simulink library "Batteries"  (R2025b)
settings: Solver=VariableStepAuto  StartTime=0.0  StopTime=10.0  RelTol=1e-3
undefined symbols (not defined in the file or in its folder): battery_builder_rtmsupport, gcbh
libraries: Batteries_lib x12
(part 2 of 2)

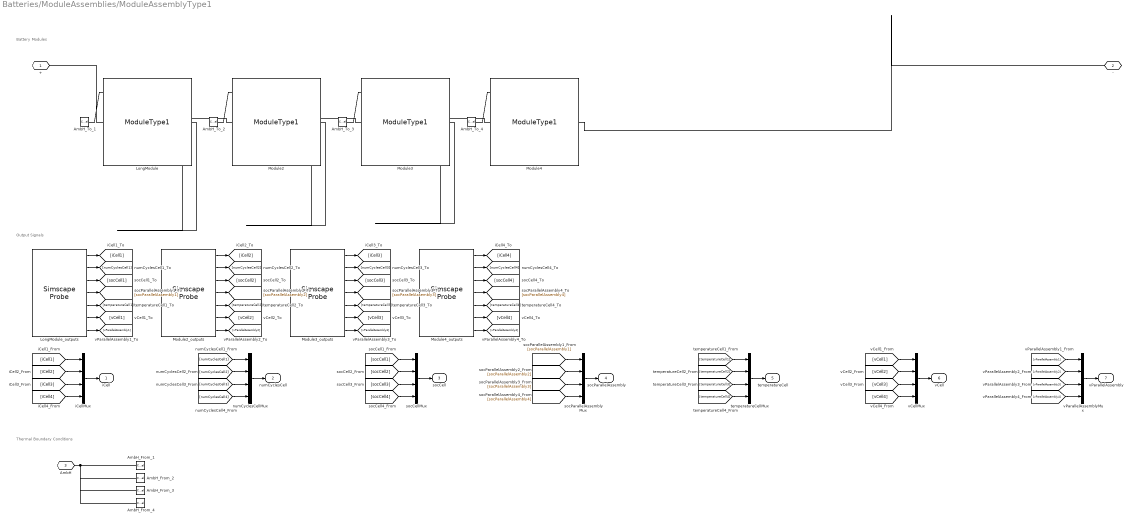
== system Batteries/ModuleAssemblies/ModuleAssemblyType1 ==
  note: Battery Modules
  note: Output Signals
  note: Thermal Boundary Conditions
  AmbH_From_1 : ConnectionLabel  Label=ambH_1
  AmbH_From_2 : ConnectionLabel  Label=ambH_2
  AmbH_From_3 : ConnectionLabel  Label=ambH_3
  AmbH_From_4 : ConnectionLabel  Label=ambH_4
  AmbH_To_1 : ConnectionLabel  Label=ambH_1
  AmbH_To_2 : ConnectionLabel  Label=ambH_2
  AmbH_To_3 : ConnectionLabel  Label=ambH_3
  AmbH_To_4 : ConnectionLabel  Label=ambH_4
  LongModule : Batteries_lib/Modules/ModuleType1  SOC_vecCell=[0, .1, .25, .5, .75, .9, 1]  T_vecCell=[278, 293, 313] K  V0_matCell=[3.49, 3.5, 3.51; 3.55, 3.57, 3.56; 3.62, 3.63, 3.64; 3.71, 3.71, 3.72; 3.91, 3.93, 3.94; 4.07, 4.08, 4.08; 4.19, 4.19, 4.19] V  V_rangeCell=[0, inf] V  R0_matCell=[.0117, .0085, .009; .011, .0085, .009; .0114, .0087, .0092; .0107, .0082, .0088; .0107, .0083, .0091; .0113, .0085, .0089; .0116, .0085, .0089] Ohm  AHCell=27 A*hr  extrapolation_optionCell=simscape.enum.extrapolation.nearest  thermal_massCell=100 J/K  CoolantResistance=1.2 K/W  AmbientResistance=25 K/W  P=20  S=2  iCell_specify=off  iCell_priority=None  iCell=0 A  iCell_nominal_specify=off  iCell_nominal_value=1  iCell_nominal_unit=A  vCell_specify=off  vCell_priority=None  vCell=0 V  vCell_nominal_specify=off  vCell_nominal_value=1  vCell_nominal_unit=V  socCell_specify=off  socCell_priority=High  socCell=1  socCell_nominal_specify=off  socCell_nominal_value=1  socCell_nominal_unit=1  numCyclesCell_specify=off  numCyclesCell_priority=High  numCyclesCell=0  numCyclesCell_nominal_specify=off  numCyclesCell_nominal_value=1  numCyclesCell_nominal_unit=1  temperatureCell_specify=off  temperatureCell_priority=High  temperatureCell=298.15 K  temperatureCell_nominal_specify=off  temperatureCell_nominal_value=1  temperatureCell_nominal_unit=K  vParallelAssembly_specify=off  vParallelAssembly_priority=None  vParallelAssembly=repmat(0, 2, 1) V  vParallelAssembly_nominal_specify=off  vParallelAssembly_nominal_value=1  vParallelAssembly_nominal_unit=V  socParallelAssembly_specify=off  socParallelAssembly_priority=None  socParallelAssembly=repmat(1, 2, 1)  socParallelAssembly_nominal_specify=off  socParallelAssembly_nominal_value=1  socParallelAssembly_nominal_unit=1
      settings: InternalSimscapePortConfiguration="{\"Bottom\":[{\"id\":\"n\",\"label\":\"-\",\"type\":\"foundation.electrical.electrical\"}],\"Left\":[{\"id\":\"AmbH\",\"label\":\"AmbH\",\"type\":\"foundation.thermal.thermal\"}],\"Right\":[],\"Top\":[{\"id\":\"p\",\"label\":\"+\",\"type\":\"foundation.electrical.electrical\"},{\"id\":\"TopExtClnt\",\"label\":\"CPT\",\"type\":\"foundation.thermal.thermal\"}]}"
  LongModule_outputs : SimscapeProbe  BoundBlock=3  Variables="{\"iCell\":{\"Probing\":\"ON\"},\"numCyclesCell\":{\"Probing\":\"ON\"},\"socCell\":{\"Probing\":\"ON\"},\"socParallelAssembly\":{\"Probing\":\"ON\"},\"temperatureCell\":{\"Probing\":\"ON\"},\"vCell\":{\"Probing\":\"ON\"},\"vParallelAssembly\":{\"Probing\":\"ON\"}}"
  Module2 : Batteries_lib/Modules/ModuleType1  SOC_vecCell=[0, .1, .25, .5, .75, .9, 1]  T_vecCell=[278, 293, 313] K  V0_matCell=[3.49, 3.5, 3.51; 3.55, 3.57, 3.56; 3.62, 3.63, 3.64; 3.71, 3.71, 3.72; 3.91, 3.93, 3.94; 4.07, 4.08, 4.08; 4.19, 4.19, 4.19] V  V_rangeCell=[0, inf] V  R0_matCell=[.0117, .0085, .009; .011, .0085, .009; .0114, .0087, .0092; .0107, .0082, .0088; .0107, .0083, .0091; .0113, .0085, .0089; .0116, .0085, .0089] Ohm  AHCell=27 A*hr  extrapolation_optionCell=simscape.enum.extrapolation.nearest  thermal_massCell=100 J/K  CoolantResistance=1.2 K/W  AmbientResistance=25 K/W  P=20  S=2  iCell_specify=off  iCell_priority=None  iCell=0 A  iCell_nominal_specify=off  iCell_nominal_value=1  iCell_nominal_unit=A  vCell_specify=off  vCell_priority=None  vCell=0 V  vCell_nominal_specify=off  vCell_nominal_value=1  vCell_nominal_unit=V  socCell_specify=off  socCell_priority=High  socCell=1  socCell_nominal_specify=off  socCell_nominal_value=1  socCell_nominal_unit=1  numCyclesCell_specify=off  numCyclesCell_priority=High  numCyclesCell=0  numCyclesCell_nominal_specify=off  numCyclesCell_nominal_value=1  numCyclesCell_nominal_unit=1  temperatureCell_specify=off  temperatureCell_priority=High  temperatureCell=298.15 K  temperatureCell_nominal_specify=off  temperatureCell_nominal_value=1  temperatureCell_nominal_unit=K  vParallelAssembly_specify=off  vParallelAssembly_priority=None  vParallelAssembly=repmat(0, 2, 1) V  vParallelAssembly_nominal_specify=off  vParallelAssembly_nominal_value=1  vParallelAssembly_nominal_unit=V  socParallelAssembly_specify=off  socParallelAssembly_priority=None  socParallelAssembly=repmat(1, 2, 1)  socParallelAssembly_nominal_specify=off  socParallelAssembly_nominal_value=1  socParallelAssembly_nominal_unit=1
      settings: InternalSimscapePortConfiguration="{\"Bottom\":[{\"id\":\"n\",\"label\":\"-\",\"type\":\"foundation.electrical.electrical\"}],\"Left\":[{\"id\":\"AmbH\",\"label\":\"AmbH\",\"type\":\"foundation.thermal.thermal\"}],\"Right\":[],\"Top\":[{\"id\":\"p\",\"label\":\"+\",\"type\":\"foundation.electrical.electrical\"},{\"id\":\"TopExtClnt\",\"label\":\"CPT\",\"type\":\"foundation.thermal.thermal\"}]}"
  Module2_outputs : SimscapeProbe  BoundBlock=4  Variables="{\"iCell\":{\"Probing\":\"ON\"},\"numCyclesCell\":{\"Probing\":\"ON\"},\"socCell\":{\"Probing\":\"ON\"},\"socParallelAssembly\":{\"Probing\":\"ON\"},\"temperatureCell\":{\"Probing\":\"ON\"},\"vCell\":{\"Probing\":\"ON\"},\"vParallelAssembly\":{\"Probing\":\"ON\"}}"
  Module3 : Batteries_lib/Modules/ModuleType1  SOC_vecCell=[0, .1, .25, .5, .75, .9, 1]  T_vecCell=[278, 293, 313] K  V0_matCell=[3.49, 3.5, 3.51; 3.55, 3.57, 3.56; 3.62, 3.63, 3.64; 3.71, 3.71, 3.72; 3.91, 3.93, 3.94; 4.07, 4.08, 4.08; 4.19, 4.19, 4.19] V  V_rangeCell=[0, inf] V  R0_matCell=[.0117, .0085, .009; .011, .0085, .009; .0114, .0087, .0092; .0107, .0082, .0088; .0107, .0083, .0091; .0113, .0085, .0089; .0116, .0085, .0089] Ohm  AHCell=27 A*hr  extrapolation_optionCell=simscape.enum.extrapolation.nearest  thermal_massCell=100 J/K  CoolantResistance=1.2 K/W  AmbientResistance=25 K/W  P=20  S=2  iCell_specify=off  iCell_priority=None  iCell=0 A  iCell_nominal_specify=off  iCell_nominal_value=1  iCell_nominal_unit=A  vCell_specify=off  vCell_priority=None  vCell=0 V  vCell_nominal_specify=off  vCell_nominal_value=1  vCell_nominal_unit=V  socCell_specify=off  socCell_priority=High  socCell=1  socCell_nominal_specify=off  socCell_nominal_value=1  socCell_nominal_unit=1  numCyclesCell_specify=off  numCyclesCell_priority=High  numCyclesCell=0  numCyclesCell_nominal_specify=off  numCyclesCell_nominal_value=1  numCyclesCell_nominal_unit=1  temperatureCell_specify=off  temperatureCell_priority=High  temperatureCell=298.15 K  temperatureCell_nominal_specify=off  temperatureCell_nominal_value=1  temperatureCell_nominal_unit=K  vParallelAssembly_specify=off  vParallelAssembly_priority=None  vParallelAssembly=repmat(0, 2, 1) V  vParallelAssembly_nominal_specify=off  vParallelAssembly_nominal_value=1  vParallelAssembly_nominal_unit=V  socParallelAssembly_specify=off  socParallelAssembly_priority=None  socParallelAssembly=repmat(1, 2, 1)  socParallelAssembly_nominal_specify=off  socParallelAssembly_nominal_value=1  socParallelAssembly_nominal_unit=1
      settings: InternalSimscapePortConfiguration="{\"Bottom\":[{\"id\":\"n\",\"label\":\"-\",\"type\":\"foundation.electrical.electrical\"}],\"Left\":[{\"id\":\"AmbH\",\"label\":\"AmbH\",\"type\":\"foundation.thermal.thermal\"}],\"Right\":[],\"Top\":[{\"id\":\"p\",\"label\":\"+\",\"type\":\"foundation.electrical.electrical\"},{\"id\":\"TopExtClnt\",\"label\":\"CPT\",\"type\":\"foundation.thermal.thermal\"}]}"
  Module3_outputs : SimscapeProbe  BoundBlock=5  Variables="{\"iCell\":{\"Probing\":\"ON\"},\"numCyclesCell\":{\"Probing\":\"ON\"},\"socCell\":{\"Probing\":\"ON\"},\"socParallelAssembly\":{\"Probing\":\"ON\"},\"temperatureCell\":{\"Probing\":\"ON\"},\"vCell\":{\"Probing\":\"ON\"},\"vParallelAssembly\":{\"Probing\":\"ON\"}}"
  Module4 : Batteries_lib/Modules/ModuleType1  SOC_vecCell=[0, .1, .25, .5, .75, .9, 1]  T_vecCell=[278, 293, 313] K  V0_matCell=[3.49, 3.5, 3.51; 3.55, 3.57, 3.56; 3.62, 3.63, 3.64; 3.71, 3.71, 3.72; 3.91, 3.93, 3.94; 4.07, 4.08, 4.08; 4.19, 4.19, 4.19] V  V_rangeCell=[0, inf] V  R0_matCell=[.0117, .0085, .009; .011, .0085, .009; .0114, .0087, .0092; .0107, .0082, .0088; .0107, .0083, .0091; .0113, .0085, .0089; .0116, .0085, .0089] Ohm  AHCell=27 A*hr  extrapolation_optionCell=simscape.enum.extrapolation.nearest  thermal_massCell=100 J/K  CoolantResistance=1.2 K/W  AmbientResistance=25 K/W  P=20  S=2  iCell_specify=off  iCell_priority=None  iCell=0 A  iCell_nominal_specify=off  iCell_nominal_value=1  iCell_nominal_unit=A  vCell_specify=off  vCell_priority=None  vCell=0 V  vCell_nominal_specify=off  vCell_nominal_value=1  vCell_nominal_unit=V  socCell_specify=off  socCell_priority=High  socCell=1  socCell_nominal_specify=off  socCell_nominal_value=1  socCell_nominal_unit=1  numCyclesCell_specify=off  numCyclesCell_priority=High  numCyclesCell=0  numCyclesCell_nominal_specify=off  numCyclesCell_nominal_value=1  numCyclesCell_nominal_unit=1  temperatureCell_specify=off  temperatureCell_priority=High  temperatureCell=298.15 K  temperatureCell_nominal_specify=off  temperatureCell_nominal_value=1  temperatureCell_nominal_unit=K  vParallelAssembly_specify=off  vParallelAssembly_priority=None  vParallelAssembly=repmat(0, 2, 1) V  vParallelAssembly_nominal_specify=off  vParallelAssembly_nominal_value=1  vParallelAssembly_nominal_unit=V  socParallelAssembly_specify=off  socParallelAssembly_priority=None  socParallelAssembly=repmat(1, 2, 1)  socParallelAssembly_nominal_specify=off  socParallelAssembly_nominal_value=1  socParallelAssembly_nominal_unit=1
      settings: InternalSimscapePortConfiguration="{\"Bottom\":[{\"id\":\"n\",\"label\":\"-\",\"type\":\"foundation.electrical.electrical\"}],\"Left\":[{\"id\":\"AmbH\",\"label\":\"AmbH\",\"type\":\"foundation.thermal.thermal\"}],\"Right\":[],\"Top\":[{\"id\":\"p\",\"label\":\"+\",\"type\":\"foundation.electrical.electrical\"},{\"id\":\"TopExtClnt\",\"label\":\"CPT\",\"type\":\"foundation.thermal.thermal\"}]}"
  Module4_outputs : SimscapeProbe  BoundBlock=6  Variables="{\"iCell\":{\"Probing\":\"ON\"},\"numCyclesCell\":{\"Probing\":\"ON\"},\"socCell\":{\"Probing\":\"ON\"},\"socParallelAssembly\":{\"Probing\":\"ON\"},\"temperatureCell\":{\"Probing\":\"ON\"},\"vCell\":{\"Probing\":\"ON\"},\"vParallelAssembly\":{\"Probing\":\"ON\"}}"
  iCellMux : Mux
  numCyclesCellMux : Mux
  socCellMux : Mux
  socParallelAssemblyMux : Mux
  temperatureCellMux : Mux
  vCellMux : Mux
  vParallelAssemblyMux : Mux
  + : PMIOPort  Side=Left
  - : PMIOPort  Port=2  Side=Right
  AmbH : PMIOPort  Port=3  Side=Right  ConnectionType=Connection: foundation.thermal.thermal
  iCell : Outport
  numCyclesCell : Outport  Port=2
  socCell : Outport  Port=3
  socParallelAssembly : Outport  Port=4
  temperatureCell : Outport  Port=5
  vCell : Outport  Port=6
  vParallelAssembly : Outport  Port=7
  wires:
  LongModule_outputs/1 -> [iCell1]
  iCellMux/1 -> iCell/1
  [iCell1] -> iCellMux/1
  LongModule_outputs/2 -> [numCyclesCell1]
  numCyclesCellMux/1 -> numCyclesCell/1
  [numCyclesCell1] -> numCyclesCellMux/1
  LongModule_outputs/3 -> [socCell1]
  socCellMux/1 -> socCell/1
  [socCell1] -> socCellMux/1
  LongModule_outputs/4 -> [socParallelAssembly1]
  socParallelAssemblyMux/1 -> socParallelAssembly/1
  [socParallelAssembly1] -> socParallelAssemblyMux/1
  LongModule_outputs/5 -> [temperatureCell1]
  temperatureCellMux/1 -> temperatureCell/1
  [temperatureCell1] -> temperatureCellMux/1
  LongModule_outputs/6 -> [vCell1]
  vCellMux/1 -> vCell/1
  [vCell1] -> vCellMux/1
  LongModule_outputs/7 -> [vParallelAssembly1]
  vParallelAssemblyMux/1 -> vParallelAssembly/1
  [vParallelAssembly1] -> vParallelAssemblyMux/1
  Module2_outputs/1 -> [iCell2]
  [iCell2] -> iCellMux/2
  Module2_outputs/2 -> [numCyclesCell2]
  [numCyclesCell2] -> numCyclesCellMux/2
  Module2_outputs/3 -> [socCell2]
  [socCell2] -> socCellMux/2
  Module2_outputs/4 -> [socParallelAssembly2]
  [socParallelAssembly2] -> socParallelAssemblyMux/2
  Module2_outputs/5 -> [temperatureCell2]
  [temperatureCell2] -> temperatureCellMux/2
  Module2_outputs/6 -> [vCell2]
  [vCell2] -> vCellMux/2
  Module2_outputs/7 -> [vParallelAssembly2]
  [vParallelAssembly2] -> vParallelAssemblyMux/2
  Module3_outputs/1 -> [iCell3]
  [iCell3] -> iCellMux/3
  Module3_outputs/2 -> [numCyclesCell3]
  [numCyclesCell3] -> numCyclesCellMux/3
  Module3_outputs/3 -> [socCell3]
  [socCell3] -> socCellMux/3
  Module3_outputs/4 -> [socParallelAssembly3]
  [socParallelAssembly3] -> socParallelAssemblyMux/3
  Module3_outputs/5 -> [temperatureCell3]
  [temperatureCell3] -> temperatureCellMux/3
  Module3_outputs/6 -> [vCell3]
  [vCell3] -> vCellMux/3
  Module3_outputs/7 -> [vParallelAssembly3]
  [vParallelAssembly3] -> vParallelAssemblyMux/3
  Module4_outputs/1 -> [iCell4]
  [iCell4] -> iCellMux/4
  Module4_outputs/2 -> [numCyclesCell4]
  [numCyclesCell4] -> numCyclesCellMux/4
  Module4_outputs/3 -> [socCell4]
  [socCell4] -> socCellMux/4
  Module4_outputs/4 -> [socParallelAssembly4]
  [socParallelAssembly4] -> socParallelAssemblyMux/4
  Module4_outputs/5 -> [temperatureCell4]
  [temperatureCell4] -> temperatureCellMux/4
  Module4_outputs/6 -> [vCell4]
  [vCell4] -> vCellMux/4
  Module4_outputs/7 -> [vParallelAssembly4]
  [vParallelAssembly4] -> vParallelAssemblyMux/4
  connections:
  Module2/LConn2 -- LongModule/RConn1
  Module3/LConn2 -- Module2/RConn1
  Module4/LConn2 -- Module3/RConn1
  LongModule/LConn2 -- +/RConn1
  Module4/RConn1 -- -/RConn1
  AmbH_To_1/LConn1 -- LongModule/LConn1
  AmbH_From_1/LConn1 -- AmbH_From_2/LConn1 -- AmbH_From_3/LConn1 -- AmbH/RConn1 -- AmbH_From_4/LConn1
  AmbH_To_2/LConn1 -- Module2/LConn1
  AmbH_To_3/LConn1 -- Module3/LConn1
  AmbH_To_4/LConn1 -- Module4/LConn1
